simulink model "q_aero_2dof_lqr_control"  (R2025a)
settings: Solver=ode1  StartTime=0.0  StopTime=30  FixedStep=0.002  RelTol=1e-3  EnableMultiTasking=on
PreLoadFcn:
  | quanser_aero_lqr
undefined symbols (not defined in the file or in its folder): K
libraries: simulink_extras x4, quarc_library x3, quanser_aero x1
settings Model: SimulationMode=external  ExtModeTrigDuration=15000  Creator=MLevis  LastModifiedBy=najem1u
settings SolverCC: AlgebraicLoopSolver=TrustRegion  PositivePriorityOrder=on
settings DataIOCC: LimitDataPoints=on  SaveFormat=Array  ReturnWorkspaceOutputs=off
settings DebuggingCC: SolverPrmCheckMsg=warning  UnconnectedInputMsg=warning  UnconnectedOutputMsg=warning  UnconnectedLineMsg=warning  SFUnexpectedBacktrackingDiag=warning  SFNoUnconditionalDefaultTransitionDiag=warning  SFExecutionAtInitializationDiag=none  ArithmeticOperatorsInVariantConditions=warning
settings ModelReferenceCC: PropagateSignalLabelsOutOfModel=off
settings SFSimCC: SimUseLocalCustomCode=off  CustomCodeUndefinedFunction=UseInterfaceOnly
settings RTWCC: SystemTargetFile=quarc_win64.tlc  TemplateMakefile=quarc_default_tmf  RTWUseLocalCustomCode=off  Toolchain=QUARC win64 | nmake (64-bit Windows)  BuildConfiguration=Faster Runs  GPUComputeCapability=3.5  Description=QUARC Win64 Target Using Toolchain
settings CodeAppCC: StateflowObjectComments=on
settings STFCustomTargetCC: SystemTargetFile=quarc_win64.tlc  MultiwordLength=2048.0  DynamicStringBufferSize=256.0  ConcurrentExecutionCompliant=on  UseToolchainInfoCompliant=on
settings GRTTargetCC: ExtMode=on  ExtModeMexFile=quarc_comm  TargetLangStandard=C89/C90 (ANSI)  ParMdlRefBuildCompliant=off  CompOptLevelCompliant=off  CombineOutputUpdateFcns=off  MatFileLogging=off  CPPClassGenCompliant=off  GRTInterface=on
settings ConfigComp: CovMetricSettings=dw  CovSaveCumulativeToWorkspaceVar=on  CovSaveSingleToWorkspaceVar=on  CovExternalEMLEnable=off  CovSFcnEnable=off

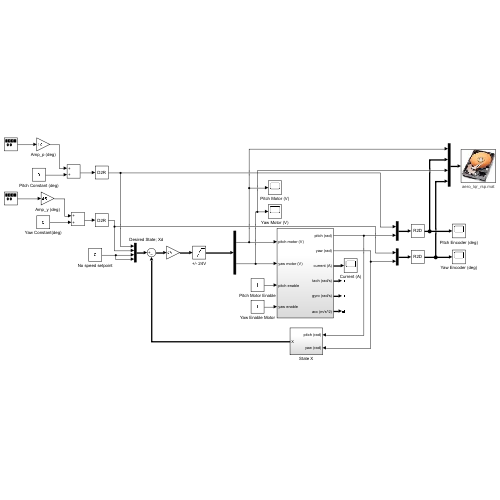
[thumbnail: Simulink's stored preview of the top-level diagram]
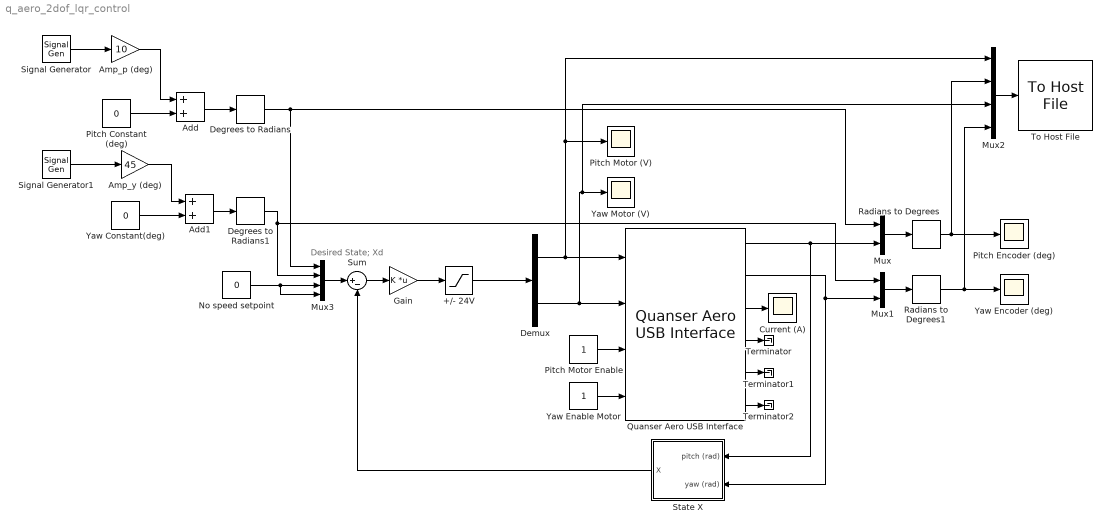
== system q_aero_2dof_lqr_control ==
  note: Desired State; Xd
  +/- 24V : Saturate  UpperLimit=24  LowerLimit=-24
  Add : Sum
  Add1 : Sum
  Amp_p (deg) : Gain  Gain=10
  Amp_y (deg) : Gain  Gain=45
  Current (A) : Scope
      settings: TimeSpan=5  DataLoggingSaveFormat=Array
  Degrees to Radians : simulink_extras/Transformations/Degrees to Radians
  Degrees to Radians1 : simulink_extras/Transformations/Degrees to Radians
  Demux : Demux  Outputs=2
  Gain : Gain  Gain=K  Multiplication=Matrix(K*u)
  Mux : Mux  Inputs=2
  Mux1 : Mux  Inputs=2
  Mux2 : Mux
  Mux3 : Mux
  No speed setpoint : Constant  Value=0
  Pitch Constant (deg) : Constant  Value=0
  Pitch Encoder (deg) : Scope
      settings: TimeSpan=30  ActiveDisplayYMinimum=-45  ActiveDisplayYMaximum=45  DataLoggingMaxPoints=15000  DataLoggingVariableName=ScopeData3  DataLoggingSaveFormat=Array
  Pitch Motor (V) : Scope
      settings: TimeSpan=30  ActiveDisplayYMinimum=-25  ActiveDisplayYMaximum=25  DataLoggingMaxPoints=15000  DataLoggingVariableName=ScopeData2  DataLoggingSaveFormat=Array
  Pitch Motor Enable : Constant
  Quanser Aero USB Interface : quanser_aero/Quanser Aero USB Interface  SystemSampleTime=-1  VariantActivationTime=update diagram  EmptyChoice=off  PassThrough=off  PassThroughVariantControl=(default)  EmptyChoiceVariantControl=(default)  AllowFlexibleInterface=on  Latency=0  AutoFrameSizeCalculation=off
  Radians to Degrees : simulink_extras/Transformations/Radians to Degrees
  Radians to Degrees1 : simulink_extras/Transformations/Radians to Degrees
  Signal Generator : SignalGenerator  WaveForm=square  Frequency=0.1
  Signal Generator1 : SignalGenerator  WaveForm=square  Frequency=0.04
  State X : Subsystem
  Sum : Sum  Inputs=|+-
  Terminator : Terminator
  Terminator1 : Terminator
  Terminator2 : Terminator
  To Host File : quarc_library/Sinks/To Host/To Host File  source=Specify via dialog (do not evaluate)  file_name=aero_lqr_rsp.mat  variable_name=lqr_rsp  decimation=1  sample_time=-1  file_format=MAT-file v.4  options=No header or footer  append=off  final_file_name=aero_lqr_rsp.mat  encoding=Default  bitrate=0
  Yaw Constant(deg) : Constant  Value=0
  Yaw Enable Motor : Constant
  Yaw Encoder (deg) : Scope
      settings: TimeSpan=30  ActiveDisplayYMinimum=-120  ActiveDisplayYMaximum=120  DataLoggingMaxPoints=15000  DataLoggingVariableName=ScopeData4  DataLoggingSaveFormat=Array
  Yaw Motor (V) : Scope
      settings: TimeSpan=30  ActiveDisplayYMinimum=-25  ActiveDisplayYMaximum=25  DataLoggingMaxPoints=15000  DataLoggingVariableName=ScopeData5  DataLoggingSaveFormat=Array
  wires:
  Degrees to Radians/1 -> Mux3/1, Mux/1
  Degrees to Radians1/1 -> Mux3/2, Mux1/1
  Signal Generator/1 -> Amp_p (deg)/1
  Pitch Constant (deg)/1 -> Add/2
  Add/1 -> Degrees to Radians/1
  Yaw Constant(deg)/1 -> Add1/2
  Amp_p (deg)/1 -> Add/1
  Signal Generator1/1 -> Amp_y (deg)/1
  Amp_y (deg)/1 -> Add1/1
  Add1/1 -> Degrees to Radians1/1
  Mux/1 -> Radians to Degrees/1
  Radians to Degrees/1 -> Mux2/2, Pitch Encoder (deg)/1
  Radians to Degrees1/1 -> Yaw Encoder (deg)/1, Mux2/4
  Pitch Motor Enable/1 -> Quanser Aero USB Interface/3
  Yaw Enable Motor/1 -> Quanser Aero USB Interface/4
  Gain/1 -> +/- 24V/1
  Demux/1 -> Quanser Aero USB Interface/1, Mux2/1, Pitch Motor (V)/1
  Demux/2 -> Quanser Aero USB Interface/2, Mux2/3, Yaw Motor (V)/1
  Sum/1 -> Gain/1
  Mux1/1 -> Radians to Degrees1/1
  Mux3/1 -> Sum/1
  No speed setpoint/1 -> Mux3/4, Mux3/3
  +/- 24V/1 -> Demux/1
  State X/1(X) -> Sum/2
  Quanser Aero USB Interface/3 -> Current (A)/1
  Quanser Aero USB Interface/1 -> Mux/2, State X/1(pitch (rad))
  Quanser Aero USB Interface/2 -> Mux1/2, State X/2(yaw (rad))
  Quanser Aero USB Interface/4 -> Terminator/1
  Quanser Aero USB Interface/5 -> Terminator1/1
  Quanser Aero USB Interface/6 -> Terminator2/1
  Mux2/1 -> To Host File/1

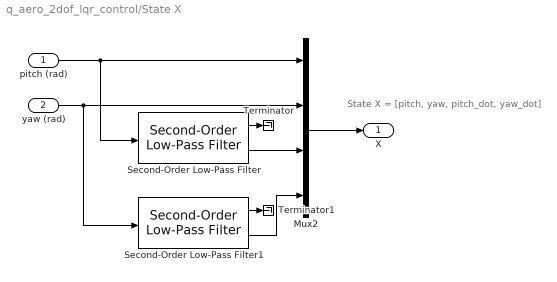
== system q_aero_2dof_lqr_control/State X ==
  note: State X = [pitch, yaw, pitch_dot, yaw_dot]
  pitch (rad) : Inport
  yaw (rad) : Inport  Port=2
  Mux2 : Mux
  Second-Order Low-Pass Filter : quarc_library/Continuous/Second-Order Low-Pass Filter  params_source=Internal (dialog parameters)  input_width=50  input_zeta=0.8  input_init=0
  Second-Order Low-Pass Filter1 : quarc_library/Continuous/Second-Order Low-Pass Filter  params_source=Internal (dialog parameters)  input_width=50  input_zeta=0.8  input_init=0
  Terminator : Terminator
  Terminator1 : Terminator
  X : Outport
  wires:
  Mux2/1 -> X/1
  yaw (rad)/1 -> Second-Order Low-Pass Filter1/1, Mux2/2
  pitch (rad)/1 -> Second-Order Low-Pass Filter/1, Mux2/1
  Second-Order Low-Pass Filter/2 -> Mux2/3
  Second-Order Low-Pass Filter1/2 -> Mux2/4
  Second-Order Low-Pass Filter/1 -> Terminator/1
  Second-Order Low-Pass Filter1/1 -> Terminator1/1
